simulink model "mdlFxPt"  (Simulink 5.2)
settings: Solver=FixedStepDiscrete  StartTime=0.0  StopTime=inf  RelTol=1e-3
PreLoadFcn:
  | mdlData;
values from neighbouring files (symbols this model uses):
  p_i16_01 = 1    [mdlData.m]
  p_i16_02 = 2    [mdlData.m]
  p_i32_01 = 1    [mdlData.m]
  p_i32_02 = 2    [mdlData.m]
  p_i8_01 = 1    [mdlData.m]
  p_i8_02 = 2    [mdlData.m]
  p_u16_01 = 1    [mdlData.m]
  p_u16_02 = 2    [mdlData.m]
  p_u32_01 = 1    [mdlData.m]
  p_u32_02 = 2    [mdlData.m]
  p_u8_01 = 1    [mdlData.m]
  p_u8_02 = 2    [mdlData.m]
libraries: lib_CATutils_Utilities_DocBlock x4, lib_CATutils_Utilities_RevNoteBlock x3, package_instance x1, lib_CATutils_Comparison_CompareToZero x1
settings Model: LastModifiedBy=KagyRA  ExtModeMexFile=no_ext_comm  SaveTime=off  SaveOutput=off  LimitDataPoints=off  ParameterPrecisionLossMsg=none  RTWInlineParameters=on  BooleanDataType=on  ProdHWDeviceType=Microprocessor  RTWSystemTargetFile=cat_ert.tlc  RTWTemplateMakefile=cat_ert_default_tmf  RTWGenerateCodeOnly=on  RTWRetainRTWFile=on  RTWOptions="-aASAP2FileDirectory=\".\" -aCAT_MaxStackSize=\"rtInf\" -aCAT_OVregexp=\"\" -aCadetWinFileDirectory=\".\" -aCatASAP2Config_MeasurementSignalGroups=\"Model_Hierarchy_Only\" -aCatASAP2Config_ModelHierarchyGroups=\"Pruned_Model_Hierarchy\" -aCatASAP2Config_SymbolNamingCompiler=\"A4_(Diab_ELF)\" -aCatCadetWinConfig_CreateArrayParameter=1 -aCatCadetWinConfig_CreateArraySignal=1 -aCatCadetWinConfig_CreateMap=1 -aCatCadetWinConfig_MID=\"0xFF\" -aCatCalToolConfig_ConvertPIDF=0 -aCatCalToolConfig_CreateASAP2=0 -aCatCalToolConfig_CreateCadetWin=0 -aCatCalToolConfig_CreateDebug=0 -aCatCalToolConfig_CreateEMC2=0 -aCatCalToolConfig_CreateGredi=0 -aCatEMC2Config_AppendInstance=1 -aCatEMC2Config_ApplyStaticVarBandAid=0 -aCatEMC2Config_CreateUnnamedVariables=0 -aCatEMC2Config_GenerateMapFile=1 -aCatEMC2Config_GenerateParFile=1 -aCatEMC2Config_GenerateRemapFcnFile=0 -aCatEMC2Config_MangleParameters=\"Add_underscore_h_to_Param_entry\" -aCatEMC2Config_NameGuidelines=\"Short_Name_Valid_in_all_Tools\" -aCatGrediConfig_BinBaseAddress=\"0x2DA000\" -aCatGrediConfig_BinSize=40 -aCatGrediConfig_CANBaudrate=250 -aCatGrediConfig_CROID=\"0x2010000\" -aCatGrediConfig_DTOID=\"0x2020000\" -aCatGrediConfig_ECUType=\"0x022D\" -aCatGrediConfig_MeasurementBaseAddress=\"0x2C0800\" -aCatGrediConfig_NodeID=\"0x0001\" -aCatGrediConfig_SampleInterval=20 -aCatGrediConfig_TID=1 -aCat_CheckForScopeDisplayBlocks=0 -aCat_RedExclmPreventCodeGen=0 -aCat_SkipEMC2GeneratedFiles=0 -aCombineOutputUpdateFcns=1 -aConfigSourceFileDirectory=\".\" -aEMC2SourceFileDirectory=\".\" -aERTCreateCustomFiles=1 -aERTCustomFileBanners=0 -aERTCustomFileTemplate=\"example_file_process.tlc\" -aERTHdrFileBannerTemplate=\"example_banner.tlc\" -aERTSrcFileBannerTemplate=\"example_banner.tlc\" -aEnforceIntegerDowncast=1 -aExtMode=0 -aExtModeTesting=0 -aFixPtUtilType=\"macro\" -aFoldNonRolledExpr=1 -aForceParamTrailComments=0 -aGenFloatMathFcnCalls=\"ANSI_C\" -aGenerateASAP2=0 -aGenerateComments=1 -aGenerateErtSFunction=0 -aGeneratePackageArchCode=\"ModelCodeAndPackageObjectFile\" -aGenerateReport=0 -aGenerateSampleERTMain=0 -aGrediFileDirectory=\".\" -aIgnoreCustomStorageClasses=0 -aIncDataTypeInIds=0 -aIncHierarchyInIds=0 -aIncludeMdlTerminateFcn=1 -aInitFltsAndDblsToZero=1 -aInlineInvariantSignals=0 -aInlineParameters=1 -aInlinedParameterPlacement=\"NonHierarchical\" -aInlinedPrmAccess=\"Literals\" -aInsertBlockDesc=0 -aLocalBlockOutputs=1 -aMapIncludeFileDirectory=\".\" -aMapSourceFileDirectory=\".\" -aMatFileLogging=0 -aMaxRTWIdLen=31 -aMultiInstanceERTCode=1 -aMultiInstanceErrorCode=\"None\" -aPackageIncludeFileDirectory=\".\" -aPackageSourceFileDirectory=\".\" -aPrefixModelToSubsysFcnNames=1 -aPurelyIntegerCode=1 -aRTWVerbose=1 -aRfdDevelopTableStructFileName=\"<DevelopTableStructFileName>\" -aRfdDevelopTableStructName=\"<DevelopTableStructName>\" -aRfdIncludeFileDirectory=\".\" -aRfdSourceFileDirectory=\".\" -aRollThreshold=5 -aRootIOStructures=0 -aShowEliminatedStatements=0 -aSpecialFilesAndDirectories=\"\" -aSuppressErrorStatus=1 -aTargetOS=\"None\" -aTuneIncludeFileDirectory=\".\" -aZeroExternalMemoryAtStartup=0 -aZeroInternalMemoryAtStartup=1"

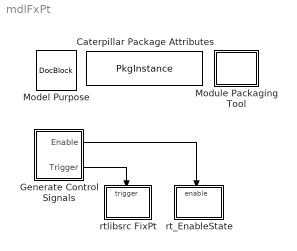
== system mdlFxPt ==
  Caterpillar Package Attributes : package_instance/PkgInstance  pkgName=mdlFxPt  InitTaskTag=SSS_TID_INIT  availModelRates={ '1.000', 'SSS_TID_1005MSEC'; '0.12', 'SSS_TID_120MSEC'; }
  Generate Control Signals : Subsystem
  Model Purpose : lib_CATutils_Utilities_DocBlock/DocBlock  isHTML=off
  Module Packaging Tool : Subsystem  Description=MPM
      settings: AttributesFormatString=Module\nPackaging\nTool\n  CopyFcn=mcb('mdlFxPt')  ModelCloseFcn=mpm_callback('MPTClose',[])  PreSaveFcn=set_param(gcb, 'CopyFcn', ['mcb(''', bdroot, ''')']);  OpenFcn=mpm_gui_options(bdroot)
      mask Type: ModulePackagingTool
      mask Description: This is the Module Packaging Tool
      mask Display: image(imread('mpm_icon.bmp','bmp'))
  rt_EnableState : Subsystem
  rtlibsrc FixPt : Subsystem
  wires:
  Generate Control Signals/2(Trigger) -> rtlibsrc FixPt/Trigger
  Generate Control Signals/1(Enable) -> rt_EnableState/Enable

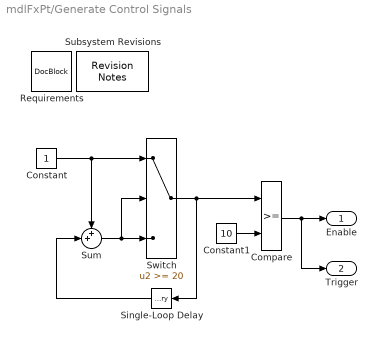
== system mdlFxPt/Generate Control Signals ==
  Compare : RelationalOperator  LogicOutDataTypeMode=Boolean  InputSameDT=on
  Constant : Constant  ShowAdditionalParam=on  OutDataTypeMode=int32  SampleTime=1
  Constant1 : Constant  Value=10  ShowAdditionalParam=on
  Requirements : lib_CATutils_Utilities_DocBlock/DocBlock  isHTML=off
  Single-Loop Delay : Memory  Orientation=left  InheritSampleTime=on
  Subsystem Revisions : lib_CATutils_Utilities_RevNoteBlock/Revision Notes  data=struct('User','---','Date',730486,'Revision','---')
  Sum : Sum  Inputs=++|  SaturateOnIntegerOverflow=on  InputSameDT=on
  Switch : Switch  Threshold=20  SaturateOnIntegerOverflow=on  InputSameDT=on
  Enable : Outport
  Trigger : Outport  Port=2
  wires:
  Constant/1 -> Switch/1, Sum/1
  Sum/1 -> Switch/3, Switch/2
  Switch/1 -> Single-Loop Delay/1, Compare/1
  Single-Loop Delay/1 -> Sum/2
  Constant1/1 -> Compare/2
  Compare/1 -> Enable/1, Trigger/1

== system mdlFxPt/Module Packaging Tool ==
  Subsystem : Subsystem

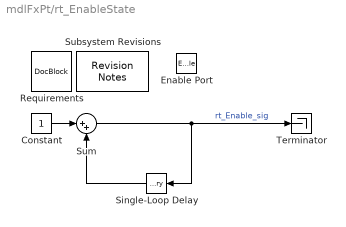
== system mdlFxPt/rt_EnableState ==
  Enable Port : EnablePort  StatesWhenEnabling=reset
  Constant : Constant  ShowAdditionalParam=on  OutDataTypeMode=uint32
  Requirements : lib_CATutils_Utilities_DocBlock/DocBlock  isHTML=off
  Single-Loop Delay : Memory  Orientation=left  InheritSampleTime=on
  Subsystem Revisions : lib_CATutils_Utilities_RevNoteBlock/Revision Notes  data=struct('User','---','Date',730486,'Revision','---')
  Sum : Sum  Inputs=|++  ShowAdditionalParam=on  SaturateOnIntegerOverflow=on  InputSameDT=on
  Terminator : Terminator
  wires:
  Constant/1 -> Sum/1
  Single-Loop Delay/1 -> Sum/2
  Sum/1 -> Single-Loop Delay/1, Terminator/1  "rt_Enable_sig"

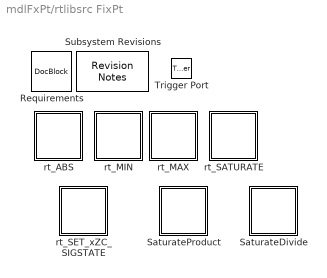
== system mdlFxPt/rtlibsrc FixPt ==
  Trigger Port : TriggerPort  TriggerType=either
  Requirements : lib_CATutils_Utilities_DocBlock/DocBlock  isHTML=off
  SaturateDivide : Subsystem
  SaturateProduct : Subsystem
  Subsystem Revisions : lib_CATutils_Utilities_RevNoteBlock/Revision Notes  data=struct('User','---','Date',730486,'Revision','---')
  rt_ABS : Subsystem
  rt_MAX : Subsystem
  rt_MIN : Subsystem
  rt_SATURATE : Subsystem
  rt_SET_xZC_SIGSTATE : Subsystem

== system mdlFxPt/Module Packaging Tool/Subsystem ==

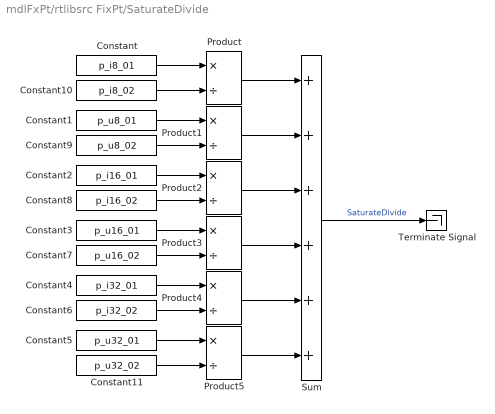
== system mdlFxPt/rtlibsrc FixPt/SaturateDivide ==
  Constant : Constant  Value=p_i8_01  ShowAdditionalParam=on  OutDataTypeMode=int8
  Constant1 : Constant  Value=p_u8_01  ShowAdditionalParam=on  OutDataTypeMode=uint8
  Constant10 : Constant  Value=p_i8_02  ShowAdditionalParam=on
  Constant11 : Constant  Value=p_u32_02  ShowAdditionalParam=on
  Constant2 : Constant  Value=p_i16_01  ShowAdditionalParam=on  OutDataTypeMode=int16
  Constant3 : Constant  Value=p_u16_01  ShowAdditionalParam=on  OutDataTypeMode=uint16
  Constant4 : Constant  Value=p_i32_01  ShowAdditionalParam=on  OutDataTypeMode=int32
  Constant5 : Constant  Value=p_u32_01  ShowAdditionalParam=on  OutDataTypeMode=uint32
  Constant6 : Constant  Value=p_i32_02  ShowAdditionalParam=on
  Constant7 : Constant  Value=p_u16_02  ShowAdditionalParam=on
  Constant8 : Constant  Value=p_i16_02  ShowAdditionalParam=on
  Constant9 : Constant  Value=p_u8_02  ShowAdditionalParam=on
  Product{,1..5} (6 alike) : Product  Inputs=*/  ShowAdditionalParam=on  SaturateOnIntegerOverflow=on  InputSameDT=on
  Sum : Sum  Inputs=6  ShowAdditionalParam=on  OutDataTypeMode=uint32  SaturateOnIntegerOverflow=on
  Terminate Signal : Terminator
  wires:
  Sum/1 -> Terminate Signal/1  "SaturateDivide"
  Constant/1 -> Product/1
  Constant10/1 -> Product/2
  Constant1/1 -> Product1/1
  Constant2/1 -> Product2/1
  Constant3/1 -> Product3/1
  Constant4/1 -> Product4/1
  Constant5/1 -> Product5/1
  Constant9/1 -> Product1/2
  Constant8/1 -> Product2/2
  Constant7/1 -> Product3/2
  Constant6/1 -> Product4/2
  Constant11/1 -> Product5/2
  Product/1 -> Sum/1
  Product1/1 -> Sum/2
  Product2/1 -> Sum/3
  Product3/1 -> Sum/4
  Product4/1 -> Sum/5
  Product5/1 -> Sum/6

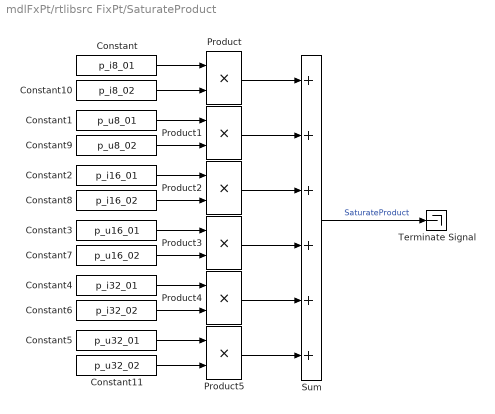
== system mdlFxPt/rtlibsrc FixPt/SaturateProduct ==
  Constant : Constant  Value=p_i8_01  ShowAdditionalParam=on  OutDataTypeMode=int8
  Constant1 : Constant  Value=p_u8_01  ShowAdditionalParam=on  OutDataTypeMode=uint8
  Constant10 : Constant  Value=p_i8_02  ShowAdditionalParam=on
  Constant11 : Constant  Value=p_u32_02  ShowAdditionalParam=on
  Constant2 : Constant  Value=p_i16_01  ShowAdditionalParam=on  OutDataTypeMode=int16
  Constant3 : Constant  Value=p_u16_01  ShowAdditionalParam=on  OutDataTypeMode=uint16
  Constant4 : Constant  Value=p_i32_01  ShowAdditionalParam=on  OutDataTypeMode=int32
  Constant5 : Constant  Value=p_u32_01  ShowAdditionalParam=on  OutDataTypeMode=uint32
  Constant6 : Constant  Value=p_i32_02  ShowAdditionalParam=on
  Constant7 : Constant  Value=p_u16_02  ShowAdditionalParam=on
  Constant8 : Constant  Value=p_i16_02  ShowAdditionalParam=on
  Constant9 : Constant  Value=p_u8_02  ShowAdditionalParam=on
  Product{,1..5} (6 alike) : Product  ShowAdditionalParam=on  SaturateOnIntegerOverflow=on  InputSameDT=on
  Sum : Sum  Inputs=6  ShowAdditionalParam=on  OutDataTypeMode=uint32  SaturateOnIntegerOverflow=on
  Terminate Signal : Terminator
  wires:
  Product5/1 -> Sum/6
  Product4/1 -> Sum/5
  Product3/1 -> Sum/4
  Product2/1 -> Sum/3
  Product1/1 -> Sum/2
  Product/1 -> Sum/1
  Constant11/1 -> Product5/2
  Constant6/1 -> Product4/2
  Constant7/1 -> Product3/2
  Constant8/1 -> Product2/2
  Constant9/1 -> Product1/2
  Constant5/1 -> Product5/1
  Constant4/1 -> Product4/1
  Constant3/1 -> Product3/1
  Constant2/1 -> Product2/1
  Constant1/1 -> Product1/1
  Constant10/1 -> Product/2
  Constant/1 -> Product/1
  Sum/1 -> Terminate Signal/1  "SaturateProduct"

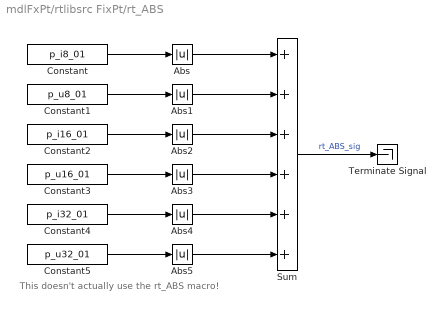
== system mdlFxPt/rtlibsrc FixPt/rt_ABS ==
  note: This doesn't actually use the
      | rt_ABS macro!
  Abs{,1..5} (6 alike) : Abs  SaturateOnIntegerOverflow=on
  Constant : Constant  Value=p_i8_01  ShowAdditionalParam=on  OutDataTypeMode=int8
  Constant1 : Constant  Value=p_u8_01  ShowAdditionalParam=on  OutDataTypeMode=uint8
  Constant2 : Constant  Value=p_i16_01  ShowAdditionalParam=on  OutDataTypeMode=int16
  Constant3 : Constant  Value=p_u16_01  ShowAdditionalParam=on  OutDataTypeMode=uint16
  Constant4 : Constant  Value=p_i32_01  ShowAdditionalParam=on  OutDataTypeMode=int32
  Constant5 : Constant  Value=p_u32_01  ShowAdditionalParam=on  OutDataTypeMode=uint32
  Sum : Sum  Inputs=6  ShowAdditionalParam=on  OutDataTypeMode=uint32  SaturateOnIntegerOverflow=on
  Terminate Signal : Terminator
  wires:
  Constant/1 -> Abs/1
  Abs/1 -> Sum/1
  Sum/1 -> Terminate Signal/1  "rt_ABS_sig"
  Constant1/1 -> Abs1/1
  Abs1/1 -> Sum/2
  Constant2/1 -> Abs2/1
  Constant3/1 -> Abs3/1
  Constant4/1 -> Abs4/1
  Constant5/1 -> Abs5/1
  Abs2/1 -> Sum/3
  Abs3/1 -> Sum/4
  Abs4/1 -> Sum/5
  Abs5/1 -> Sum/6

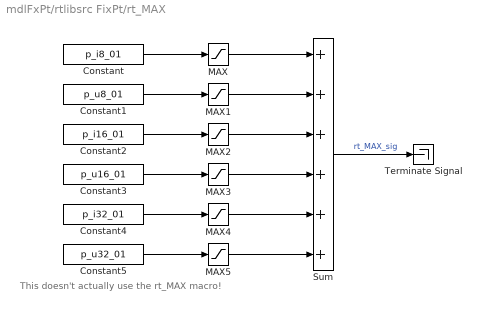
== system mdlFxPt/rtlibsrc FixPt/rt_MAX ==
  note: This doesn't actually use the
      | rt_MAX macro!
  Constant : Constant  Value=p_i8_01  ShowAdditionalParam=on  OutDataTypeMode=int8
  Constant1 : Constant  Value=p_u8_01  ShowAdditionalParam=on  OutDataTypeMode=uint8
  Constant2 : Constant  Value=p_i16_01  ShowAdditionalParam=on  OutDataTypeMode=int16
  Constant3 : Constant  Value=p_u16_01  ShowAdditionalParam=on  OutDataTypeMode=uint16
  Constant4 : Constant  Value=p_i32_01  ShowAdditionalParam=on  OutDataTypeMode=int32
  Constant5 : Constant  Value=p_u32_01  ShowAdditionalParam=on  OutDataTypeMode=uint32
  MAX : Saturate  UpperLimit=9  LowerLimit=int8(-inf)
  MAX1 : Saturate  UpperLimit=9  LowerLimit=uint8(-inf)
  MAX2 : Saturate  UpperLimit=9  LowerLimit=int16(-inf)
  MAX3 : Saturate  UpperLimit=9  LowerLimit=uint16(-inf)
  MAX4 : Saturate  UpperLimit=9  LowerLimit=int32(-inf)
  MAX5 : Saturate  UpperLimit=9  LowerLimit=uint32(-inf)
  Sum : Sum  Inputs=6  ShowAdditionalParam=on  OutDataTypeMode=uint32  SaturateOnIntegerOverflow=on
  Terminate Signal : Terminator
  wires:
  Constant/1 -> MAX/1
  MAX/1 -> Sum/1
  Sum/1 -> Terminate Signal/1  "rt_MAX_sig"
  Constant1/1 -> MAX1/1
  MAX1/1 -> Sum/2
  Constant2/1 -> MAX2/1
  Constant3/1 -> MAX3/1
  Constant4/1 -> MAX4/1
  Constant5/1 -> MAX5/1
  MAX2/1 -> Sum/3
  MAX3/1 -> Sum/4
  MAX4/1 -> Sum/5
  MAX5/1 -> Sum/6

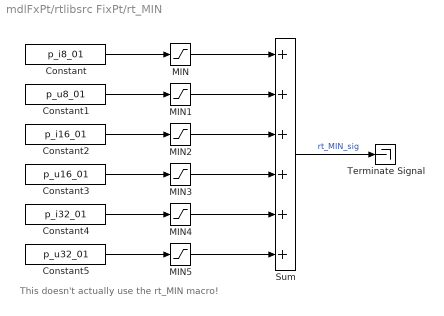
== system mdlFxPt/rtlibsrc FixPt/rt_MIN ==
  note: This doesn't actually use the
      | rt_MIN macro!
  Constant : Constant  Value=p_i8_01  ShowAdditionalParam=on  OutDataTypeMode=int8
  Constant1 : Constant  Value=p_u8_01  ShowAdditionalParam=on  OutDataTypeMode=uint8
  Constant2 : Constant  Value=p_i16_01  ShowAdditionalParam=on  OutDataTypeMode=int16
  Constant3 : Constant  Value=p_u16_01  ShowAdditionalParam=on  OutDataTypeMode=uint16
  Constant4 : Constant  Value=p_i32_01  ShowAdditionalParam=on  OutDataTypeMode=int32
  Constant5 : Constant  Value=p_u32_01  ShowAdditionalParam=on  OutDataTypeMode=uint32
  MIN : Saturate  UpperLimit=int8(inf)  LowerLimit=3
  MIN1 : Saturate  UpperLimit=uint8(inf)  LowerLimit=3
  MIN2 : Saturate  UpperLimit=int16(inf)  LowerLimit=3
  MIN3 : Saturate  UpperLimit=uint16(inf)  LowerLimit=3
  MIN4 : Saturate  UpperLimit=int32(inf)  LowerLimit=3
  MIN5 : Saturate  UpperLimit=uint32(inf)  LowerLimit=3
  Sum : Sum  Inputs=6  ShowAdditionalParam=on  OutDataTypeMode=uint32  SaturateOnIntegerOverflow=on
  Terminate Signal : Terminator
  wires:
  MIN5/1 -> Sum/6
  MIN4/1 -> Sum/5
  MIN3/1 -> Sum/4
  MIN2/1 -> Sum/3
  Constant5/1 -> MIN5/1
  Constant4/1 -> MIN4/1
  Constant3/1 -> MIN3/1
  Constant2/1 -> MIN2/1
  MIN1/1 -> Sum/2
  Constant1/1 -> MIN1/1
  Sum/1 -> Terminate Signal/1  "rt_MIN_sig"
  MIN/1 -> Sum/1
  Constant/1 -> MIN/1

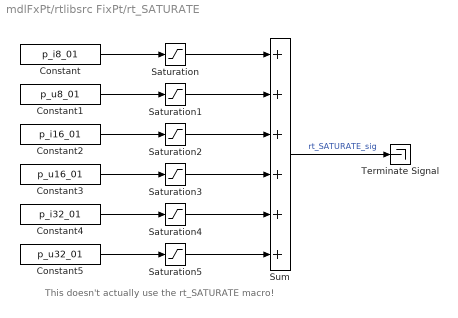
== system mdlFxPt/rtlibsrc FixPt/rt_SATURATE ==
  note: This doesn't actually use the
      | rt_SATURATE macro!
  Constant : Constant  Value=p_i8_01  ShowAdditionalParam=on  OutDataTypeMode=int8
  Constant1 : Constant  Value=p_u8_01  ShowAdditionalParam=on  OutDataTypeMode=uint8
  Constant2 : Constant  Value=p_i16_01  ShowAdditionalParam=on  OutDataTypeMode=int16
  Constant3 : Constant  Value=p_u16_01  ShowAdditionalParam=on  OutDataTypeMode=uint16
  Constant4 : Constant  Value=p_i32_01  ShowAdditionalParam=on  OutDataTypeMode=int32
  Constant5 : Constant  Value=p_u32_01  ShowAdditionalParam=on  OutDataTypeMode=uint32
  Saturation{,1..5} (6 alike) : Saturate  UpperLimit=9  LowerLimit=3
  Sum : Sum  Inputs=6  ShowAdditionalParam=on  OutDataTypeMode=uint32  SaturateOnIntegerOverflow=on
  Terminate Signal : Terminator
  wires:
  Saturation5/1 -> Sum/6
  Saturation4/1 -> Sum/5
  Saturation3/1 -> Sum/4
  Saturation2/1 -> Sum/3
  Constant5/1 -> Saturation5/1
  Constant4/1 -> Saturation4/1
  Constant3/1 -> Saturation3/1
  Constant2/1 -> Saturation2/1
  Saturation1/1 -> Sum/2
  Constant1/1 -> Saturation1/1
  Sum/1 -> Terminate Signal/1  "rt_SATURATE_sig"
  Saturation/1 -> Sum/1
  Constant/1 -> Saturation/1

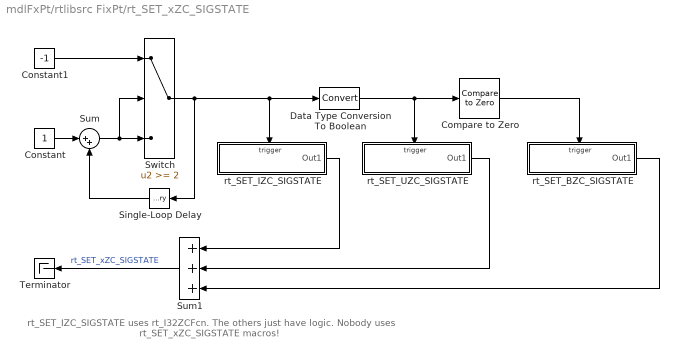
== system mdlFxPt/rtlibsrc FixPt/rt_SET_xZC_SIGSTATE ==
  note: rt_SET_IZC_SIGSTATE uses rt_I32ZCFcn.  The others just have logic.
      | Nobody uses rt_SET_xZC_SIGSTATE macros!
  Compare to Zero : lib_CATutils_Comparison_CompareToZero/Compare to Zero  relop=~=  outDT=Boolean
  Constant : Constant  ShowAdditionalParam=on
  Constant1 : Constant  Value=-1  ShowAdditionalParam=on  OutDataTypeMode=int8
  Data Type Conversion To Boolean : DataTypeConversion  DataType=uint8  SaturateOnIntegerOverflow=on
  Single-Loop Delay : Memory  Orientation=left  InheritSampleTime=on
  Sum : Sum  Inputs=|++  SaturateOnIntegerOverflow=on  InputSameDT=on
  Sum1 : Sum  Orientation=left  Inputs=3  ShowAdditionalParam=on  SaturateOnIntegerOverflow=on  InputSameDT=on
  Switch : Switch  Threshold=2  SaturateOnIntegerOverflow=on  InputSameDT=on
  Terminator : Terminator
  rt_SET_BZC_SIGSTATE : Subsystem  TreatAsAtomicUnit=on
  rt_SET_IZC_SIGSTATE : Subsystem  TreatAsAtomicUnit=on
  rt_SET_UZC_SIGSTATE : Subsystem  TreatAsAtomicUnit=on
  wires:
  Constant/1 -> Sum/1
  Sum/1 -> Switch/3, Switch/2
  Switch/1 -> Single-Loop Delay/1, rt_SET_IZC_SIGSTATE/Trigger, Data Type Conversion To Boolean/1
  Single-Loop Delay/1 -> Sum/2
  Constant1/1 -> Switch/1
  rt_SET_IZC_SIGSTATE/1(Out1) -> Sum1/1
  rt_SET_UZC_SIGSTATE/1(Out1) -> Sum1/2
  Data Type Conversion To Boolean/1 -> rt_SET_UZC_SIGSTATE/Trigger, Compare to Zero/1
  Compare to Zero/1 -> rt_SET_BZC_SIGSTATE/Trigger
  rt_SET_BZC_SIGSTATE/1(Out1) -> Sum1/3
  Sum1/1 -> Terminator/1  "rt_SET_xZC_SIGSTATE"

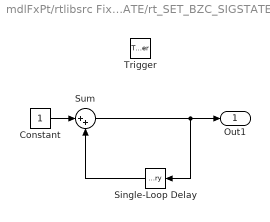
== system mdlFxPt/rtlibsrc FixPt/rt_SET_xZC_SIGSTATE/rt_SET_BZC_SIGSTATE ==
  Trigger : TriggerPort  TriggerType=either
  Constant : Constant  ShowAdditionalParam=on  OutDataTypeMode=uint32
  Single-Loop Delay : Memory  Orientation=left  InheritSampleTime=on
  Sum : Sum  Inputs=|++  ShowAdditionalParam=on  SaturateOnIntegerOverflow=on  InputSameDT=on
  Out1 : Outport
  wires:
  Constant/1 -> Sum/1
  Single-Loop Delay/1 -> Sum/2
  Sum/1 -> Single-Loop Delay/1, Out1/1

== system mdlFxPt/rtlibsrc FixPt/rt_SET_xZC_SIGSTATE/rt_SET_IZC_SIGSTATE ==
  Trigger : TriggerPort  TriggerType=either
  Constant : Constant  ShowAdditionalParam=on  OutDataTypeMode=uint32
  Single-Loop Delay : Memory  Orientation=left  InheritSampleTime=on
  Sum : Sum  Inputs=|++  ShowAdditionalParam=on  SaturateOnIntegerOverflow=on  InputSameDT=on
  Out1 : Outport
  wires:
  Constant/1 -> Sum/1
  Single-Loop Delay/1 -> Sum/2
  Sum/1 -> Single-Loop Delay/1, Out1/1

== system mdlFxPt/rtlibsrc FixPt/rt_SET_xZC_SIGSTATE/rt_SET_UZC_SIGSTATE ==
  Trigger : TriggerPort  TriggerType=either
  Constant : Constant  ShowAdditionalParam=on  OutDataTypeMode=uint32
  Single-Loop Delay : Memory  Orientation=left  InheritSampleTime=on
  Sum : Sum  Inputs=|++  ShowAdditionalParam=on  SaturateOnIntegerOverflow=on  InputSameDT=on
  Out1 : Outport
  wires:
  Sum/1 -> Out1/1, Single-Loop Delay/1
  Single-Loop Delay/1 -> Sum/2
  Constant/1 -> Sum/1
